simulink model "commhdlQPSKTxRxLoopback"  (R2025b)
settings: Solver=FixedStepDiscrete  StartTime=0.0  StopTime=0.03  RelTol=1e-3
PostLoadFcn:
  | hScopeConfig = get_param([gcs '/Receiver/QPSK Rx/Frequency and Time Synchronizer/Symbol Synchronizer/No HDL/QPSK Receiver Eye Diagram'],'ScopeConfiguration');
  | 
  | hScopeConfig.OpenAtSimulationStart = false;
  | hScopeConfig.Visible = false;
  | SamplesPerSymbol = 4;
  | %UpsamplesRx = 1;
  | clear hScopeConfig
InitFcn:
  | % RxAlign decoder latency (flat_simfix): 41 = netlist value used for HDL; set
  | % rxAlignLat = 25 in the base workspace before a model-level simulation.
  | if ~exist('rxAlignLat','var'), rxAlignLat = uint16(41); end
  | commhdlQPSKTxRxModelInit;
  | % Rate bridge: ADRV9002/Jupiter radio runs at 15.36 MHz = 2x the 7.68 MHz
  | % (4 samples/symbol @ Rsym=1.92 MHz) the QPSK Rx requires. The deployed
  | % Receiver must downsample the ADC stream by 2. UpsamplesRx=1 fed the QPSK
  | % Rx 8 sps (2x-upsampled) and broke symbol sync / the loopback bit check.
  | UpsamplesRx = 1;   %% T8 RATE FIX: rail 15.36e6 == ADC bus rate,
  | %% no ingress decimation (was 2 when the rail sat on the 7.68e6 rung)
  | UpsamplesTx = 1;
  | clear simTimingOffset;
StopFcn:
  | if exist('simTimingOffset','var')
  |   disp('Simulation completed');
  |   %QPSKTxRxVerification;
  | end
undefined symbols (not defined in the file or in its folder): Add, Config, fsym, randsrc, RandStream, Rsym, rxAlignLat, Shift
libraries: hdlsllib x141, simulink x45, dspsigops x30, dsphdlfiltering2 x6, dsphdlsigops2 x4, dsphdlmathfun2 x4, commdigbbndpm3 x4, dspmlti4 x2, commchan3 x1, commrflib2 x1, commcnvcod2 x1
(part 2 of 9)

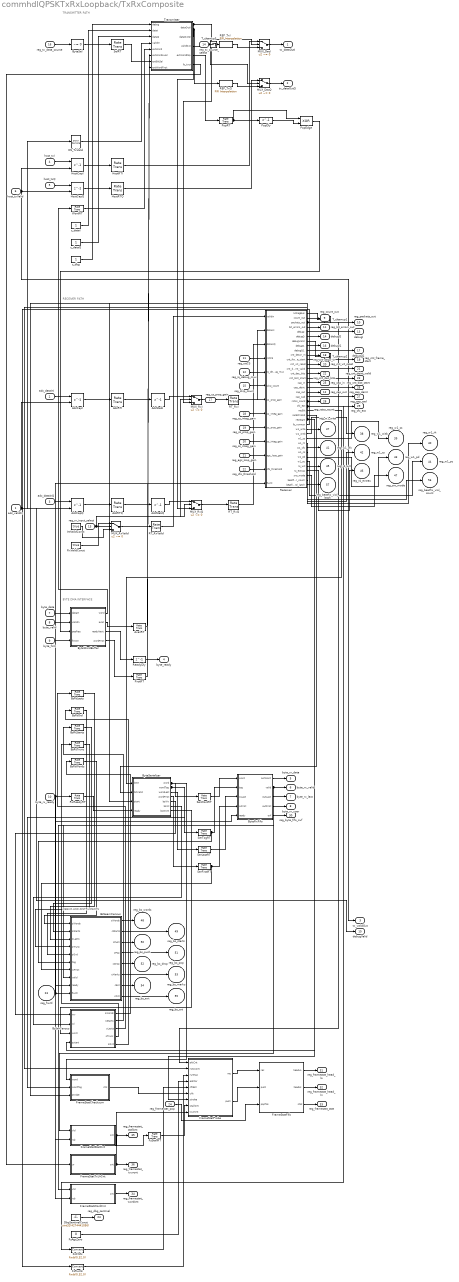
== system commhdlQPSKTxRxLoopback/TxRxComposite ==
  note: TRANSMITTER PATH
  note: RECEIVER PATH
  note: BYTE DMA INTERFACE
  note: DEBUG AND INSTRUMENTS
  adc_validIn : Inport  OutDataTypeStr=boolean  SampleTime=1/30.72e6
  adc_dataInI : Inport  Port=2  OutDataTypeStr=int16  SampleTime=1/30.72e6
  adc_dataInQ : Inport  Port=3  OutDataTypeStr=int16  SampleTime=1/30.72e6
  host_txI : Inport  Port=4  OutDataTypeStr=int16  SampleTime=1/30.72e6
  host_txQ : Inport  Port=5  OutDataTypeStr=int16  SampleTime=1/30.72e6
  host_txValid : Inport  Port=6  OutDataTypeStr=boolean  SampleTime=1/30.72e6
  byte_data : Inport  Port=7  OutDataTypeStr=uint64  SampleTime=1/30.72e6
  byte_valid : Inport  Port=8  OutDataTypeStr=boolean  SampleTime=1/30.72e6
  byte_first : Inport  Port=9  OutDataTypeStr=boolean  SampleTime=1/30.72e6
  byte_rx_ready : Inport  Port=10  OutDataTypeStr=boolean  SampleTime=1/30.72e6
  reg_rstCS : Inport  Port=11  OutDataTypeStr=boolean  SampleTime=1/15.36e6
  reg_iq_debug_mux : Inport  Port=12  OutDataTypeStr=uint32  SampleTime=1/15.36e6
  reg_rx_input_select : Inport  Port=13  OutDataTypeStr=boolean  SampleTime=1/15.36e6
  reg_tx_source_select : Inport  Port=14  OutDataTypeStr=uint32  SampleTime=1/15.36e6
  reg_skip_count : Inport  Port=15  OutDataTypeStr=uint32  SampleTime=1/15.36e6
  reg_tx_data_source : Inport  Port=16  OutDataTypeStr=uint32  SampleTime=1/15.36e6
  reg_cs_prop_gain : Inport  Port=17  OutDataTypeStr=uint32  SampleTime=1/15.36e6
  reg_cs_integ_gain : Inport  Port=18  OutDataTypeStr=uint32  SampleTime=1/15.36e6
  reg_ss_prop_gain : Inport  Port=19  OutDataTypeStr=uint32  SampleTime=1/15.36e6
  reg_ss_integ_gain : Inport  Port=20  OutDataTypeStr=uint32  SampleTime=1/15.36e6
  reg_agc_loop_gain : Inport  Port=21  OutDataTypeStr=uint32  SampleTime=1/15.36e6
  reg_cfo_threshold : Inport  Port=22  OutDataTypeStr=uint32  SampleTime=1/15.36e6
  reg_fixctl : Inport  Port=23  OutDataTypeStr=uint32
  reg_framestat_pop : Inport  Port=24  OutDataTypeStr=uint32  SampleTime=1/15.36e6
  AdcCapI : Delay  DelayLength=1  ShowEnablePort=on
      settings: InputPortMap=u0,e6
  AdcCapQ : Delay  DelayLength=1  ShowEnablePort=on
      settings: InputPortMap=u0,e6
  AdcRTI : RateTransition  OutPortSampleTime=1/15.36e6
  AdcRTQ : RateTransition  OutPortSampleTime=1/15.36e6
  AdcStabI : Delay  DelayLength=1
  AdcStabQ : Delay  DelayLength=1
  AvailRT : RateTransition  OutPortSampleTime=1/15.36e6
  BsRtLasts : RateTransition  OutPortSampleTime=1/30.72e6
  BsRtOrd : RateTransition  OutPortSampleTime=1/30.72e6
  BsRtStarts : RateTransition  OutPortSampleTime=1/30.72e6
  BsRtTrunc : RateTransition  OutPortSampleTime=1/30.72e6
  BsRtWords : RateTransition  OutPortSampleTime=1/30.72e6
  BsSeamCensus : MATLAB Function  TreatAsAtomicUnit=on
  BsSerCensus : MATLAB Function  TreatAsAtomicUnit=on
  ByteRxFifo : MATLAB Function  TreatAsAtomicUnit=on
  ByteSel : simulink/Logic and Bit Operations/Compare To Constant  relop=~=  const=0  OutDataTypeStr=boolean
  ByteSerializer : MATLAB Function  TreatAsAtomicUnit=on
  ByteWordBuffer : MATLAB Function  TreatAsAtomicUnit=on
  DS_TxValid : DownSample  N=1  RateOptions=Allow multirate processing  AllowArbitraryFixedInput=on
  DbgSentinelConst : Constant  Value=uint32(4274441056)  OutDataTypeStr=uint32  SampleTime=1/15.36e6
  FirstRT : RateTransition  OutPortSampleTime=1/15.36e6
  FrameStatChecksum : MATLAB Function  TreatAsAtomicUnit=on
  FrameStatFifo : MATLAB Function  TreatAsAtomicUnit=on
  FrameStatProbe : MATLAB Function  TreatAsAtomicUnit=on
  FrameStatStallCnt : MATLAB Function  TreatAsAtomicUnit=on
  FrameStatTxUrCnt : MATLAB Function  TreatAsAtomicUnit=on
  FrameStatWordCnt : MATLAB Function  TreatAsAtomicUnit=on
  FsAgcZero : Constant  Value=0  OutDataTypeStr=uint32
  FsCfcSi : DataTypeConversion  OutDataTypeStr=fixdt(0,32,0)  ConvertRealWorld=Stored Integer (SI)  SaturateOnIntegerOverflow=off  RndMeth=Floor
  FsRunSi : DataTypeConversion  OutDataTypeStr=fixdt(0,32,0)  ConvertRealWorld=Stored Integer (SI)  SaturateOnIntegerOverflow=off  RndMeth=Floor
  FsStallRT : RateTransition  OutPortSampleTime=1/15.36e6
  HostCapI : Delay  DelayLength=1  ShowEnablePort=on
      settings: InputPortMap=u0,e6
  HostCapQ : Delay  DelayLength=1  ShowEnablePort=on
      settings: InputPortMap=u0,e6
  HostRTI : RateTransition  OutPortSampleTime=1/30.72e6
  HostRTQ : RateTransition  OutPortSampleTime=1/30.72e6
  IntValidConst : Constant  Value=true  OutDataTypeStr=boolean  SampleTime=1/15.36e6
  MUX_DacI : Switch  Criteria=u2 ~= 0
  MUX_DacQ : Switch  Criteria=u2 ~= 0
  MUX_RxI : Switch  Criteria=u2 ~= 0
  MUX_RxQ : Switch  Criteria=u2 ~= 0
  MUX_RxValid : Switch  Criteria=u2 ~= 0
  PopDly : Delay  DelayLength=1
  PopEdge : Logic  Operator=XOR
  PopRT : RateTransition  OutPortSampleTime=1/30.72e6
  REP_TxI : dspmlti4/FIR Interpolation  FilterSource=Dialog parameters  PrivateCoeffs=0  h=2*fir1(24,0.45)  L=2  FilterObject=FINTERP  framing=Allow multirate processing  outputBufInitCond=0  roundingMode=Nearest  overflowMode=on  firstCoeffDataTypeStr=Inherit: Same word length as input  firstCoeffMin=[]  firstCoeffMax=[]  firstCoeffLastDataTypeStr=Inherit: Same word length as input  outputMin=[]  outputMax=[]
  REP_TxQ : dspmlti4/FIR Interpolation  FilterSource=Dialog parameters  PrivateCoeffs=0  h=2*fir1(24,0.45)  L=2  FilterObject=FINTERP  framing=Allow multirate processing  outputBufInitCond=0  roundingMode=Nearest  overflowMode=on  firstCoeffDataTypeStr=Inherit: Same word length as input  firstCoeffMin=[]  firstCoeffMax=[]  firstCoeffLastDataTypeStr=Inherit: Same word length as input  outputMin=[]  outputMax=[]
  RT_RxI : RateTransition  OutPortSampleTime=1/15.36e6
  RT_RxQ : RateTransition  OutPortSampleTime=1/15.36e6
  RT_RxValid : RateTransition  OutPortSampleTime=1/15.36e6
  ReadyDly : Delay  DelayLength=1  InitialCondition=1
  Receiver : Subsystem  TreatAsAtomicUnit=on
  RxReadyRT : RateTransition  OutPortSampleTime=1/15.36e6
  RxValidConst : Constant  Value=true  OutDataTypeStr=boolean  SampleTime=1/15.36e6
  SelRT : RateTransition  OutPortSampleTime=1/15.36e6
  SerFirstRT : RateTransition  OutPortSampleTime=1/30.72e6
  SerLastRT : RateTransition  OutPortSampleTime=1/30.72e6
  SerTogRT : RateTransition  OutPortSampleTime=1/30.72e6
  SerWordRT : RateTransition  OutPortSampleTime=1/30.72e6
  T_cleanup1 : Terminator
  T_cleanup2 : Terminator
  T_cleanup3 : Terminator
  Transmitter : Subsystem  TreatAsAtomicUnit=on
  WordRT : RateTransition  OutPortSampleTime=1/15.36e6
  c_dataI : Constant  OutDataTypeStr=int16  SampleTime=1/15.36e6
  c_dataQ : Constant  OutDataTypeStr=int16  SampleTime=1/15.36e6
  c_dbg : Constant  OutDataTypeStr=uint32  SampleTime=1/15.36e6
  tx_dataOutI : Outport
  tx_dataOutQ : Outport  Port=2
  tx_validOut : Outport  Port=3
  byte_ready : Outport  Port=4
  byte_rx_data : Outport  Port=5
  byte_rx_valid : Outport  Port=6
  byte_rx_last : Outport  Port=7
  byte_rx_user : Outport  Port=8
  reg_count_out : Outport  Port=9
  reg_packets_out : Outport  Port=10
  reg_bit_errors_out : Outport  Port=11
  reg_cap_out : Outport  Port=12
  debugI : Outport  Port=13
  debugQ : Outport  Port=14
  debugValid : Outport  Port=15
  debugI1 : Outport  Port=16
  debugQ1 : Outport  Port=17
  reg_cnt_descr_in : Outport  Port=18
  reg_cnt_frame_start : Outport  Port=19
  reg_cnt_vit_reset : Outport  Port=20
  reg_cnt_deint_valid : Outport  Port=21
  reg_cnt_dec_bits : Outport  Port=22
  reg_cnt_bist_start : Outport  Port=23
  reg_dbg_sentinel : Outport  Port=24
  reg_cap_in : Outport  Port=25
  reg_cap_deint : Outport  Port=26
  reg_cap_cad : Outport  Port=27
  reg_rstcs_count : Outport  Port=28
  reg_cfc_est : Outport  Port=29
  reg_byte_fifo_ovf : Outport  Port=30
  reg_framestat_head_lo : Outport  Port=31
  reg_framestat_head_hi : Outport  Port=32
  reg_framestat_stat : Outport  Port=33
  reg_framestat_wordcnt : Outport  Port=34
  reg_framestat_stallcnt : Outport  Port=35
  reg_framestat_txurcnt : Outport  Port=36
  reg_w1_wita : Outport  Port=37
  reg_w1_witb : Outport  Port=38
  reg_w1_ss : Outport  Port=39
  reg_w1_rh : Outport  Port=40
  reg_w1_cfc : Outport  Port=41
  reg_w1_cs : Outport  Port=42
  reg_w1_pd : Outport  Port=43
  reg_w1_pc : Outport  Port=44
  reg_r4_wit : Outport  Port=45
  reg_r4_extras : Outport  Port=46
  reg_sro_mode : Outport  Port=47
  reg_bs_words : Outport  Port=48
  reg_bs_starts : Outport  Port=49
  reg_bs_push : Outport  Port=50
  reg_bs_pop : Outport  Port=51
  reg_bs_drop : Outport  Port=52
  reg_bs_marks : Outport  Port=53
  reg_bs_evt : Outport  Port=54
  reg_bs_cnt : Outport  Port=55
  reg_beatfix_viol_count : Outport  Port=56
  reg_beatfix_viol_latch : Outport  Port=57
  wires:
  Receiver/30(w1_cfc) -> reg_w1_cfc/1
  BsSeamCensus/5(cDrop) -> reg_bs_drop/1
  FrameStatProbe/1(rec) -> FrameStatFifo/1(rec)
  host_txI/1 -> HostCapI/1
  MUX_RxValid/1 -> RT_RxValid/1
  Receiver/23(recBitValid) -> ByteSerializer/2(bitValid)
  byte_first/1 -> ByteWordBuffer/4(firstIn)
  AdcCapI/1 -> AdcRTI/1
  ByteSerializer/2(wordTog) -> FrameStatChecksum/2(wordTog), SerTogRT/1
  c_dataQ/1 -> Transmitter/3(dataQ)
  ByteRxFifo/3(outLast) -> byte_rx_last/1
  ReadyDly/1 -> byte_ready/1
  ByteRxFifo/5(ovf) -> reg_byte_fifo_ovf/1
  host_txValid/1 -> HostCapQ/2, HostCapI/2, tx_validOut/1
  BsRtTrunc/1 -> BsSeamCensus/4(sTrunc)
  DbgSentinelConst/1 -> reg_dbg_sentinel/1
  MUX_DacQ/1 -> tx_dataOutQ/1
  BsSeamCensus/4(cPop) -> reg_bs_pop/1
  AdcStabI/1 -> MUX_RxI/1
  BsSeamCensus/8(cCnt) -> reg_bs_cnt/1
  reg_tx_data_source/1 -> ByteSel/1
  AvailRT/1 -> Transmitter/6(extWordAvail)
  IntValidConst/1 -> MUX_RxValid/3
  Receiver/9(debugQ1) -> debugQ1/1
  adc_dataInI/1 -> AdcCapI/1
  ByteSerializer/3(wordLast) -> SerLastRT/1
  SerWordRT/1 -> ByteRxFifo/1(word)
  FrameStatWordCnt/1(cnt) -> reg_framestat_wordcnt/1
  Receiver/33(w1_pc) -> reg_w1_pc/1
  Receiver/29(w1_rh) -> reg_w1_rh/1
  reg_cs_integ_gain/1 -> Receiver/8(cs_integ_gain)
  Receiver/4(bit_errors_out) -> reg_bit_errors_out/1
  MUX_RxI/1 -> RT_RxI/1
  REP_TxI/1 -> MUX_DacI/3
  AdcRTQ/1 -> AdcStabQ/1
  Receiver/11(cnt_frame_start) -> reg_cnt_frame_start/1
  FrameStatTxUrCnt/1(cnt) -> reg_framestat_txurcnt/1, FrameStatProbe/9(txurCnt)
  Receiver/14(cnt_dec_bits) -> reg_cnt_dec_bits/1
  RT_RxI/1 -> Receiver/2(dataInI)
  Receiver/24(recStart) -> BsSerCensus/4(sstart), ByteSerializer/3(start), FrameStatProbe/7(strobe), FrameStatChecksum/3(strobe)
  Receiver/37(beatfix_viol_count) -> reg_beatfix_viol_count/1
  PopEdge/1 -> ByteWordBuffer/3(popReq)
  FrameStatFifo/1(headLo) -> reg_framestat_head_lo/1
  Receiver/38(beatfix_viol_latch) -> reg_beatfix_viol_latch/1
  Receiver/8(debugI1) -> debugI1/1
  Receiver/19(cap_cad) -> reg_cap_cad/1
  Receiver/15(cnt_bist_start) -> reg_cnt_bist_start/1
  BsSeamCensus/2(cStarts) -> reg_bs_starts/1
  byte_valid/1 -> ByteWordBuffer/2(validIn)
  reg_ss_prop_gain/1 -> Receiver/9(ss_prop_gain)
  HostRTQ/1 -> MUX_DacQ/1
  HostCapQ/1 -> HostRTQ/1
  Transmitter/4(extWordPop) -> PopRT/1
  BsSerCensus/3(sLasts) -> BsRtLasts/1
  Receiver/17(cap_deint) -> reg_cap_deint/1
  Receiver/21(cfc_est) -> FsCfcSi/1, reg_cfc_est/1
  BsSerCensus/1(sWords) -> BsRtWords/1
  MUX_RxQ/1 -> RT_RxQ/1
  Receiver/6(debugQ) -> debugQ/1
  Transmitter/1(dataOutI) -> REP_TxI/1, MUX_RxI/3
  RxValidConst/1 -> MUX_RxValid/1
  FrameStatChecksum/1(chk) -> FrameStatProbe/6(chk)
  SerTogRT/1 -> ByteRxFifo/2(tog), BsSeamCensus/6(tog)
  Receiver/34(r4_wit) -> reg_r4_wit/1
  Receiver/16(cap_in) -> reg_cap_in/1
  Receiver/31(w1_cs) -> reg_w1_cs/1
  ByteSel/1 -> SelRT/1
  Receiver/22(recBit) -> ByteSerializer/1(bitIn)
  Receiver/18(cap_out) -> reg_cap_out/1
  Receiver/26(w1_wita) -> reg_w1_wita/1
  DS_TxValid/1 -> Transmitter/4(validIn)
  ByteSerializer/6(bsWl) -> BsSerCensus/2(wl)
  FsCfcSi/1 -> FrameStatProbe/5(cfcEst)
  ByteSerializer/4(wordFirst) -> SerFirstRT/1
  FrameStatStallCnt/1(cnt) -> reg_framestat_stallcnt/1, FsStallRT/1
  FirstRT/1 -> Transmitter/8(extWordFirst)
  RT_RxQ/1 -> Receiver/3(dataInQ)
  Receiver/27(w1_witb) -> reg_w1_witb/1
  Receiver/3(packets_out) -> FrameStatProbe/1(pktCnt), reg_packets_out/1
  Receiver/10(cnt_descr_in) -> reg_cnt_descr_in/1
  reg_ss_integ_gain/1 -> Receiver/10(ss_integ_gain)
  Receiver/2(count_out) -> reg_count_out/1
  reg_skip_count/1 -> Receiver/6(skip_count)
  byte_rx_ready/1 -> RxReadyRT/1, FrameStatWordCnt/2(rdy), ByteRxFifo/5(ready), FrameStatStallCnt/2(rdy), BsSeamCensus/9(ready)
  SerFirstRT/1 -> ByteRxFifo/4(wFirst), BsSeamCensus/7(wFirst)
  HostCapI/1 -> HostRTI/1
  BsRtOrd/1 -> BsSeamCensus/5(sOrd)
  adc_dataInQ/1 -> AdcCapQ/1
  Receiver/32(w1_pd) -> reg_w1_pd/1
  reg_cs_prop_gain/1 -> Receiver/7(cs_prop_gain)
  PopRT/1 -> PopDly/1, PopEdge/1
  BsSerCensus/2(sStarts) -> BsRtStarts/1
  Receiver/20(rstcs_count) -> reg_rstcs_count/1, FrameStatProbe/2(rstcsCnt)
  FsRunSi/1 -> FrameStatProbe/3(runMax)
  reg_fixctl/1 -> BsSeamCensus/10(fixctl), Receiver/13(fixctl)
  BsRtWords/1 -> BsSeamCensus/1(sWords)
  FrameStatProbe/2(push) -> FrameStatFifo/2(push)
  BsSeamCensus/3(cPush) -> reg_bs_push/1
  MUX_DacI/1 -> tx_dataOutI/1
  SelRT/1 -> Transmitter/7(extBitSel)
  reg_framestat_pop/1 -> FrameStatFifo/3(popTok)
  FrameStatFifo/2(headHi) -> reg_framestat_head_hi/1
  Receiver/35(r4_extras) -> reg_r4_extras/1
  ByteRxFifo/4(outFirst) -> byte_rx_user/1
  REP_TxQ/1 -> MUX_DacQ/3
  reg_cfo_threshold/1 -> Receiver/12(cfo_threshold)
  Receiver/25(fs_runmax) -> FsRunSi/1
  Receiver/12(cnt_vit_reset) -> reg_cnt_vit_reset/1
  reg_agc_loop_gain/1 -> Receiver/11(agc_loop_gain)
  Transmitter/2(dataOutQ) -> REP_TxQ/1, MUX_RxQ/3
  reg_tx_source_select/1 -> MUX_DacI/2, MUX_DacQ/2
  RxReadyRT/1 -> ByteSerializer/4(ready)
  Transmitter/5(fs_txur) -> FrameStatTxUrCnt/1(ur)
  reg_rstCS/1 -> Receiver/4(rstCS)
  SerLastRT/1 -> ByteRxFifo/3(wLast)
  BsRtStarts/1 -> BsSeamCensus/2(sStarts)
  BsSeamCensus/7(cEvt) -> reg_bs_evt/1
  PopDly/1 -> PopEdge/2
  BsRtLasts/1 -> BsSeamCensus/3(sLasts)
  host_txQ/1 -> HostCapQ/1
  ByteSerializer/7(bsWcnt) -> BsSerCensus/3(wcnt)
  c_dbg/1 -> Transmitter/1(debug)
  Receiver/5(debugI) -> debugI/1
  BsSeamCensus/1(cWords) -> reg_bs_words/1
  ByteRxFifo/2(valid) -> byte_rx_valid/1, BsSeamCensus/8(valid), FrameStatWordCnt/1(vld), FrameStatStallCnt/1(vld)
  byte_data/1 -> ByteWordBuffer/1(dataIn)
  FrameStatFifo/3(stat) -> reg_framestat_stat/1
  reg_iq_debug_mux/1 -> Receiver/5(iq_debug_mux)
  WordRT/1 -> Transmitter/5(extWord)
  ByteWordBuffer/4(wordFirst) -> FirstRT/1
  ByteSerializer/1(word) -> FrameStatChecksum/1(word), SerWordRT/1
  ByteRxFifo/1(outWord) -> byte_rx_data/1
  ByteSerializer/5(bsWv) -> BsSerCensus/1(wv)
  BsSerCensus/5(sOrd) -> BsRtOrd/1
  ByteWordBuffer/2(avail) -> AvailRT/1
  RT_RxValid/1 -> Receiver/1(validIn)
  BsSeamCensus/6(cMarks) -> reg_bs_marks/1
  adc_validIn/1 -> debugValid/1, AdcCapQ/2, DS_TxValid/1, AdcCapI/2
  HostRTI/1 -> MUX_DacI/1
  BsSerCensus/4(sTrunc) -> BsRtTrunc/1
  Receiver/36(sro_mode) -> reg_sro_mode/1
  ByteWordBuffer/1(word) -> WordRT/1
  reg_rx_input_select/1 -> MUX_RxValid/2, MUX_RxQ/2, MUX_RxI/2
  FsAgcZero/1 -> FrameStatProbe/4(adcFor)
  AdcRTI/1 -> AdcStabI/1
  AdcStabQ/1 -> MUX_RxQ/1
  ByteWordBuffer/3(readyNext) -> ReadyDly/1
  Receiver/28(w1_ss) -> reg_w1_ss/1
  AdcCapQ/1 -> AdcRTQ/1
  FsStallRT/1 -> FrameStatProbe/8(stallCnt)
  Receiver/13(cnt_deint_valid) -> reg_cnt_deint_valid/1
  c_dataI/1 -> Transmitter/2(dataI)
  Receiver/1(rxDiagBus) -> T_cleanup1/1
  Receiver/7(debugValid) -> T_cleanup2/1
  Transmitter/3(validOut) -> T_cleanup3/1

== system commhdlQPSKTxRxLoopback/Capture Tx Diagnostics/Subsystem ==
  In1 : Inport
  Enable : EnablePort
  To Workspace : ToWorkspace  VariableName=simQPSKSym  SampleTime=-1
      settings: Save2DSignal=2-D array (concatenate along first dimension)
  wires:
  In1/1 -> To Workspace/1

== system commhdlQPSKTxRxLoopback/Capture Tx Diagnostics/Subsystem1 ==
  In1 : Inport
  Enable : EnablePort
  To Workspace1 : ToWorkspace  VariableName=simTxWaveform  SampleTime=-1
      settings: Save2DSignal=2-D array (concatenate along first dimension)
  wires:
  In1/1 -> To Workspace1/1

== system commhdlQPSKTxRxLoopback/Channel/Mod 1 ==
  In1 : Inport
  Constant : Constant  SampleTime=-1
  Mod : Math  Operator=mod
  Out1 : Outport
  wires:
  Mod/1 -> Out1/1
  In1/1 -> Mod/1
  Constant/1 -> Mod/2

== system commhdlQPSKTxRxLoopback/Receiver/Capture Data Bits ==
  dataOut : Inport
  dataSrt : Inport  Port=2
  dataEnd : Inport  Port=3
  valid : Inport  Port=4
  Display : Display
  Display1 : Display
  Display2 : Display
  MATLAB Function : MATLAB Function  TreatAsAtomicUnit=on
  To Workspace : ToWorkspace  VariableName=RxOut  SampleTime=-1
      settings: Save2DSignal=2-D array (concatenate along first dimension)
  To Workspace1 : ToWorkspace  VariableName=RxOutSrt  SampleTime=-1
      settings: Save2DSignal=2-D array (concatenate along first dimension)
  To Workspace2 : ToWorkspace  VariableName=RxOutEnd  SampleTime=-1
      settings: Save2DSignal=2-D array (concatenate along first dimension)
  count_out : Outport
  packets_out : Outport  Port=2
  bit_errors_out : Outport  Port=3
  wires:
  dataOut/1 -> MATLAB Function/2(datain), To Workspace/1
  dataSrt/1 -> MATLAB Function/3(start), To Workspace1/1
  dataEnd/1 -> MATLAB Function/4(stop), To Workspace2/1
  valid/1 -> MATLAB Function/1(valid)
  MATLAB Function/1(count_out) -> count_out/1, Display/1
  MATLAB Function/2(packets_out) -> packets_out/1, Display1/1
  MATLAB Function/3(bit_errors_out) -> bit_errors_out/1, Display2/1

== system commhdlQPSKTxRxLoopback/Receiver/QPSK Rx ==
  dataIn : Inport  OutDataTypeStr=fixdt(1,16,14)  PortDimensions=1  SampleTime=1/(Rsym*SamplesPerSymbol)
      settings: SignalType=complex
  validIn : Inport  Port=2  OutDataTypeStr=boolean  PortDimensions=1  SampleTime=1/(Rsym*SamplesPerSymbol)
  rstCS : Inport  Port=3  OutDataTypeStr=boolean  PortDimensions=1
      settings: SignalType=complex
  debugMuxCtrl : Inport  Port=4  OutDataTypeStr=uint32  PortDimensions=1  SampleTime=1/(Rsym*SamplesPerSymbol)
  Automatic Gain Control : Subsystem  mask{Ref=AGCReference, LFG=AGCLoopGain}
      mask prompts: Ref "Error Detector Reference:"; LFG "Loop Filter Gain"
  Bus Creator : BusCreator  Inputs=4
  Bus Creator1 : BusCreator  Inputs=3
  Complex to Real-Imag : ComplexToRealImag
  Constant : Constant  Value=true  SampleTime=1/(Rsym*SamplesPerSymbol)
  Data Type Conversion : DataTypeConversion  OutDataTypeStr=int16  ConvertRealWorld=Stored Integer (SI)  SaturateOnIntegerOverflow=off  RndMeth=Floor
  Delay{,1..8} (9 alike) : Delay  DelayLength=1
  Frequency and Time Synchronizer : Subsystem
      settings: PortSchema="{\"entries\":[{\"content\":{\"sides\":[{\"content\":{\"connectorIds\":[\"In1\",\"In2\"]},\"type\":\"ConnectorPlacement.EquallySpacedRectSide\",\"uuid\":\"8bc6a452-5111-4806-8ca9-335cb622aea6\"},{\"content\":{\"connectorIds\":[\"Out1\",\"Out2\",\"Out3\",\"Out4\"],\"side\":\"RIGHT\"},\"type\":\"ConnectorPlacement.EquallySpacedRectSide\",\"uuid\":\"b0f43c98-f5c0-4f62-94ae-d69789942eef\"},{\"content\":{\"connectorIds\":[\"In3\",\"Out7\",\"Out8\"],\"side\":\"TOP\"},\"type\":\"ConnectorPlacement.EquallySpacedRectSide\",\"uuid\":\"427ff3b3-b896-4008-9584-d311480df763\"},{\"content\":{\"connectorIds\":[\"Out5\",\"Out6\"],\"side\":\"BOTTOM\"},\"type\":\"ConnectorPlacement.EquallySpacedRectSide\",\"uuid\":\"f704cb90-80a1-4198-8b72-e70182b45e73\"},{\"content\":{\"side\":\"HIDDEN\"},\"type\":\"ConnectorPlacement.EquallySpacedRectSide\",\"uuid\":\"f6309498-1e43-486f-b6b5-2c6570711f8e\"}]},\"type\":\"ConnectorPlacement.EquallySpacedConnector\",\"uuid\":\"f0ce492e-c9e1-4b35-98ef-84d77b696cfe\"}],\"packageUris\":[\"http://schema.mathworks.com/mf0/Connector/R2020b\"],\"version\":\"1.0\"}"
  HDL Data Descrambler : Subsystem
  Index Vector : MultiPortSwitch  DataPortOrder=Zero-based contiguous  Inputs=4  DiagnosticForDefault=None  zeroidx=on  SaturateOnIntegerOverflow=off  InputSameDT=off
  QPSK Demodulator : Subsystem
  RRC Receive Filter : dsphdlfiltering2/Discrete FIR Filter  NumeratorSource=Property  Numerator=RRCCoef  NumeratorPrototype=[]  FilterStructure=Direct form systolic  SerializationOption=Minimum number of cycles between valid input samples  NumCycles=2  NumberOfMultipliers=2  SimulateUsing=Code generation  roundingMode=Floor  overflowMode=off  CoefficientsDataTypeStr=Inherit: Same word length as input  OutputDataTypeStr=Inherit: Same word length as input  ResetInputPort=off  HDLGlobalReset=off  CoeffMultiplier=Multiplier  UseMultForPow2Coeff=on  FrameInputSymmOptim=off
  dataOut : Outport
  ctrlOut : Outport  Port=2
  rxDiagBus : Outport  Port=3
  debugIOut : Outport  Port=4
  debugQOut : Outport  Port=5
  debugValid : Outport  Port=6
  wires:
  rstCS/1 -> Frequency and Time Synchronizer/3(rstCS)
  QPSK Demodulator/1(dataOut) -> HDL Data Descrambler/1(dataIn)
  validIn/1 -> Automatic Gain Control/2(validIn)
  Automatic Gain Control/2(validOut) -> RRC Receive Filter/2
  RRC Receive Filter/1 -> Frequency and Time Synchronizer/1(dataIn)
  HDL Data Descrambler/3(endOut) -> Bus Creator1/2  "endOut"
  QPSK Demodulator/3(endOut) -> HDL Data Descrambler/3(endIn)
  Frequency and Time Synchronizer/8(normCoarseFreqEst) -> Bus Creator/2  "normCoarseFreqEst"
  Bus Creator1/1 -> ctrlOut/1
  HDL Data Descrambler/2(startOut) -> Bus Creator1/1  "startOut"
  Frequency and Time Synchronizer/3(endOut) -> QPSK Demodulator/3(endIn)
  RRC Receive Filter/2 -> Frequency and Time Synchronizer/2(validIn)
  Frequency and Time Synchronizer/7(nSynced) -> Bus Creator/1  "nSynced"
  Bus Creator/1 -> Delay/1
  Automatic Gain Control/1(dataOut) -> Delay1/1, RRC Receive Filter/1
  Frequency and Time Synchronizer/1(dataOut) -> Delay4/1, QPSK Demodulator/1(dataIn), Bus Creator/3  "QPSKConstellationPoints"
  dataIn/1 -> Automatic Gain Control/1(dataIn)
  HDL Data Descrambler/1(dataOut) -> dataOut/1
  HDL Data Descrambler/4(validOut) -> Bus Creator1/3  "validOut"
  QPSK Demodulator/2(startOut) -> HDL Data Descrambler/2(startIn)
  Frequency and Time Synchronizer/2(startOut) -> QPSK Demodulator/2(startIn)
  Frequency and Time Synchronizer/4(validOut) -> QPSK Demodulator/4(validIn), Bus Creator/4  "QPSKConstellationValid"
  QPSK Demodulator/4(validOut) -> HDL Data Descrambler/4(validIn)
  Delay/1 -> rxDiagBus/1
  Frequency and Time Synchronizer/5(postSymbolSync) -> Delay2/1
  Frequency and Time Synchronizer/6(postCarrierSync) -> Delay3/1
  debugMuxCtrl/1 -> Index Vector/1
  Complex to Real-Imag/2 -> debugQOut/1
  Complex to Real-Imag/1 -> debugIOut/1
  Data Type Conversion/1 -> Delay6/1
  Delay1/1 -> Index Vector/2
  Delay2/1 -> Index Vector/3
  Delay3/1 -> Index Vector/4
  Delay4/1 -> Index Vector/5
  Delay5/1 -> Data Type Conversion/1
  Index Vector/1 -> Delay5/1
  Delay6/1 -> Complex to Real-Imag/1
  Delay7/1 -> debugValid/1
  Delay8/1 -> Delay7/1
  Constant/1 -> Delay8/1

== system commhdlQPSKTxRxLoopback/Transmitter/Input Data ==
  enb : Inport
  reset : Inport  Port=2
  Cast To Boolean : DataTypeConversion  OutDataTypeStr=boolean  SaturateOnIntegerOverflow=off  RndMeth=Floor
  Delay : Delay  DelayLength=1
  Display : Display
  Message Generator : Subsystem
  Terminator : Terminator
  Terminator1 : Terminator
  txData : Outport
  txValid : Outport  Port=2
  msg_count_out : Outport  Port=3
  wires:
  Message Generator/4(valid) -> txValid/1
  Message Generator/1(out) -> txData/1
  enb/1 -> Message Generator/2(enable)
  Message Generator/5(count) -> Display/1
  Message Generator/2(stop) -> Delay/1
  Delay/1 -> Cast To Boolean/1
  Cast To Boolean/1 -> Message Generator/1(reset)
  reset/1 -> Terminator/1
  Message Generator/3(start) -> Terminator1/1
  Message Generator/6(msg_count_out) -> msg_count_out/1

== system commhdlQPSKTxRxLoopback/Transmitter/QPSK Tx ==
  dataIn : Inport  OutDataTypeStr=boolean  PortDimensions=1
  validIn : Inport  Port=2  OutDataTypeStr=boolean  PortDimensions=1
  Bit Packetizer : Subsystem
  Bus Creator : BusCreator  Inputs=2
  HDL Data Scrambler : Subsystem
  QPSK Modulator : Subsystem
  RRC Transmit Filter : Subsystem
  dataReady : Outport
  dataOut : Outport  Port=2
  txDiagBus : Outport  Port=3
  validOut : Outport  Port=4
  wires:
  validIn/1 -> Bit Packetizer/2(validIn)
  RRC Transmit Filter/2(validOut) -> validOut/1
  HDL Data Scrambler/1(dataOut) -> QPSK Modulator/1(dataIn)
  Bit Packetizer/1(bitsOut) -> HDL Data Scrambler/1(dataIn)
  QPSK Modulator/2(validOut) -> Bus Creator/2, RRC Transmit Filter/2(validIn)  "QPSKConstellationValid"
  dataIn/1 -> Bit Packetizer/1(dataIn)
  Bit Packetizer/3(dataEnd) -> HDL Data Scrambler/3(endIn)
  HDL Data Scrambler/2(validOut) -> QPSK Modulator/2(validIn)
  RRC Transmit Filter/1(dataOut) -> dataOut/1
  QPSK Modulator/1(dataOut) -> Bus Creator/1, RRC Transmit Filter/1(dataIn)  "QPSKConstellationPoints"
  Bit Packetizer/2(dataStart) -> HDL Data Scrambler/2(startIn)
  Bit Packetizer/5(dataReady) -> dataReady/1
  Bus Creator/1 -> txDiagBus/1
  Bit Packetizer/4(bitsValid) -> HDL Data Scrambler/4(validIn)

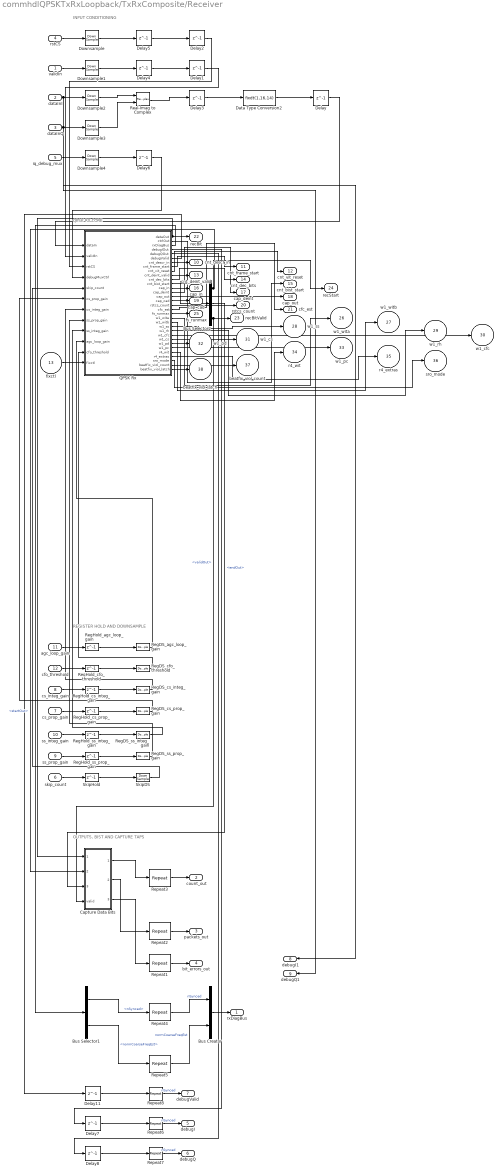
== system commhdlQPSKTxRxLoopback/TxRxComposite/Receiver ==
  note: INPUT CONDITIONING
  note: QPSK RX CORE
  note: REGISTER HOLD AND DOWNSAMPLE
  note: OUTPUTS, BIST AND CAPTURE TAPS
  validIn : Inport
  dataInI : Inport  Port=2
  dataInQ : Inport  Port=3
  rstCS : Inport  Port=4
  iq_debug_mux : Inport  Port=5  OutDataTypeStr=uint32
  skip_count : Inport  Port=6  OutDataTypeStr=uint32  SampleTime=1/15.36e6
  cs_prop_gain : Inport  Port=7  OutDataTypeStr=uint32  SampleTime=1/15.36e6
  cs_integ_gain : Inport  Port=8  OutDataTypeStr=uint32  SampleTime=1/15.36e6
  ss_prop_gain : Inport  Port=9  OutDataTypeStr=uint32  SampleTime=1/15.36e6
  ss_integ_gain : Inport  Port=10  OutDataTypeStr=uint32  SampleTime=1/15.36e6
  agc_loop_gain : Inport  Port=11  OutDataTypeStr=uint32  SampleTime=1/15.36e6
  cfo_threshold : Inport  Port=12  OutDataTypeStr=uint32  SampleTime=1/15.36e6
  fixctl : Inport  Port=13  OutDataTypeStr=uint32
  Bus Creator : BusCreator  Inputs=2
  Bus Selector1 : BusSelector  OutputSignals=nSynced,normCoarseFreqEst
  Bus Selector2 : BusSelector  OutputSignals=startOut,endOut,validOut
  Capture Data Bits : Subsystem
  Data Type Conversion2 : DataTypeConversion  OutDataTypeStr=fixdt(1,16,14)  ConvertRealWorld=Stored Integer (SI)  SaturateOnIntegerOverflow=off  RndMeth=Floor
  Delay{,1..8,11} (10 alike) : Delay  DelayLength=1
  Downsample{,1..4} (5 alike) : DownSample  N=UpsamplesRx  RateOptions=Allow multirate processing
  QPSK Rx : Subsystem
      mask init: same as commhdlQPSKTxRxLoopback/Receiver/QPSK Rx
  Real-Imag to Complex : RealImagToComplex
  RegDS_agc_loop_gain : DownSample  N=1  RateOptions=Allow multirate processing  AllowArbitraryFixedInput=on
  RegDS_cfo_threshold : DownSample  N=1  RateOptions=Allow multirate processing  AllowArbitraryFixedInput=on
  RegDS_cs_integ_gain : DownSample  N=1  RateOptions=Allow multirate processing  AllowArbitraryFixedInput=on
  RegDS_cs_prop_gain : DownSample  N=1  RateOptions=Allow multirate processing  AllowArbitraryFixedInput=on
  RegDS_ss_integ_gain : DownSample  N=1  RateOptions=Allow multirate processing  AllowArbitraryFixedInput=on
  RegDS_ss_prop_gain : DownSample  N=1  RateOptions=Allow multirate processing  AllowArbitraryFixedInput=on
  RegHold_agc_loop_gain : Delay  DelayLength=1
  RegHold_cfo_threshold : Delay  DelayLength=1
  RegHold_cs_integ_gain : Delay  DelayLength=1
  RegHold_cs_prop_gain : Delay  DelayLength=1
  RegHold_ss_integ_gain : Delay  DelayLength=1
  RegHold_ss_prop_gain : Delay  DelayLength=1
  Repeat{1..8} (8 alike) : dspsigops/Repeat  FactorSource=Dialog parameter  N=UpsamplesRx  Nmax=16  InputProcessing=Columns as channels (frame based)  RateOptions=Allow multirate processing  ic=0  mode=Unused parameter value
      settings: LibrarySourceBlock=commsequence2/Repeat
  SkipDS : DownSample  N=1  RateOptions=Allow multirate processing  AllowArbitraryFixedInput=on
  SkipHold : Delay  DelayLength=1
  rxDiagBus : Outport
  count_out : Outport  Port=2
  packets_out : Outport  Port=3
  bit_errors_out : Outport  Port=4
  debugI : Outport  Port=5
  debugQ : Outport  Port=6
  debugValid : Outport  Port=7
  debugI1 : Outport  Port=8
  debugQ1 : Outport  Port=9
  cnt_descr_in : Outport  Port=10
  cnt_frame_start : Outport  Port=11
  cnt_vit_reset : Outport  Port=12
  cnt_deint_valid : Outport  Port=13
  cnt_dec_bits : Outport  Port=14
  cnt_bist_start : Outport  Port=15
  cap_in : Outport  Port=16
  cap_deint : Outport  Port=17
  cap_out : Outport  Port=18
  cap_cad : Outport  Port=19
  rstcs_count : Outport  Port=20
  cfc_est : Outport  Port=21
  recBit : Outport  Port=22
  recBitValid : Outport  Port=23
  recStart : Outport  Port=24
  fs_runmax : Outport  Port=25
  w1_wita : Outport  Port=26
  w1_witb : Outport  Port=27
  w1_ss : Outport  Port=28
  w1_rh : Outport  Port=29
  w1_cfc : Outport  Port=30
  w1_cs : Outport  Port=31
  w1_pd : Outport  Port=32
  w1_pc : Outport  Port=33
  r4_wit : Outport  Port=34
  r4_extras : Outport  Port=35
  sro_mode : Outport  Port=36
  beatfix_viol_count : Outport  Port=37
  beatfix_viol_latch : Outport  Port=38
  wires:
  Downsample3/1 -> Real-Imag to Complex/2
  validIn/1 -> Downsample1/1
  Bus Selector2/1 -> Capture Data Bits/2(dataSrt), recStart/1  "<startOut>"
  Bus Selector2/2 -> Capture Data Bits/3(dataEnd)  "<endOut>"
  Bus Selector2/3 -> recBitValid/1, Capture Data Bits/4(valid)  "<validOut>"
  Delay3/1 -> Data Type Conversion2/1
  Delay1/1 -> QPSK Rx/2(validIn)
  Delay6/1 -> QPSK Rx/4(debugMuxCtrl)
  Downsample4/1 -> Delay6/1
  Capture Data Bits/1(count_out) -> Repeat3/1
  Capture Data Bits/2(packets_out) -> Repeat2/1
  Capture Data Bits/3(bit_errors_out) -> Repeat1/1
  Data Type Conversion2/1 -> Delay/1
  QPSK Rx/3(rxDiagBus) -> Bus Selector1/1
  QPSK Rx/1(dataOut) -> recBit/1, Capture Data Bits/1(dataOut)
  QPSK Rx/5(debugQOut) -> Delay8/1
  QPSK Rx/8(cnt_frame_start) -> cnt_frame_start/1
  QPSK Rx/9(cnt_vit_reset) -> cnt_vit_reset/1
  QPSK Rx/4(debugIOut) -> Delay7/1
  SkipDS/1 -> QPSK Rx/5(skip_count)
  RegHold_cfo_threshold/1 -> RegDS_cfo_threshold/1
  RegDS_cfo_threshold/1 -> QPSK Rx/11(cfo_threshold)
  QPSK Rx/21(w1_witb) -> w1_witb/1
  dataInQ/1 -> Downsample3/1, debugQ1/1
  QPSK Rx/14(cap_deint) -> cap_deint/1
  Bus Selector1/1 -> Repeat4/1  "<nSynced>"
  Repeat4/1 -> Bus Creator/1  "nSynced"
  iq_debug_mux/1 -> Downsample4/1
  RegHold_agc_loop_gain/1 -> RegDS_agc_loop_gain/1
  SkipHold/1 -> SkipDS/1
  RegHold_ss_prop_gain/1 -> RegDS_ss_prop_gain/1
  Bus Creator/1 -> rxDiagBus/1
  rstCS/1 -> Downsample/1
  cs_prop_gain/1 -> RegHold_cs_prop_gain/1
  Delay4/1 -> Delay1/1
  QPSK Rx/13(cap_in) -> cap_in/1
  Downsample/1 -> Delay5/1
  Delay/1 -> QPSK Rx/1(dataIn)
  ss_prop_gain/1 -> RegHold_ss_prop_gain/1
  cfo_threshold/1 -> RegHold_cfo_threshold/1
  QPSK Rx/20(w1_wita) -> w1_wita/1
  Delay7/1 -> Repeat6/1
  skip_count/1 -> SkipHold/1
  RegHold_ss_integ_gain/1 -> RegDS_ss_integ_gain/1
  QPSK Rx/22(w1_ss) -> w1_ss/1
  QPSK Rx/2(ctrlOut) -> Bus Selector2/1
  Delay8/1 -> Repeat7/1
  Delay5/1 -> Delay2/1
  Bus Selector1/2 -> Repeat5/1  "<normCoarseFreqEst>"
  QPSK Rx/12(cnt_bist_start) -> cnt_bist_start/1
  cs_integ_gain/1 -> RegHold_cs_integ_gain/1
  ss_integ_gain/1 -> RegHold_ss_integ_gain/1
  Repeat5/1 -> Bus Creator/2  "normCoarseFreqEst"
  Repeat8/1 -> debugValid/1  "nSynced"
  QPSK Rx/10(cnt_deint_valid) -> cnt_deint_valid/1
  RegHold_cs_integ_gain/1 -> RegDS_cs_integ_gain/1
  RegDS_cs_integ_gain/1 -> QPSK Rx/7(cs_integ_gain)
  RegDS_ss_prop_gain/1 -> QPSK Rx/8(ss_prop_gain)
  agc_loop_gain/1 -> RegHold_agc_loop_gain/1
  Repeat6/1 -> debugI/1  "nSynced"
  RegDS_cs_prop_gain/1 -> QPSK Rx/6(cs_prop_gain)
  QPSK Rx/29(r4_extras) -> r4_extras/1
  QPSK Rx/7(cnt_descr_in) -> cnt_descr_in/1
  fixctl/1 -> QPSK Rx/12(fixctl)
  RegDS_agc_loop_gain/1 -> QPSK Rx/10(agc_loop_gain)
  dataInI/1 -> debugI1/1, Downsample2/1
  Real-Imag to Complex/1 -> Delay3/1
  RegDS_ss_integ_gain/1 -> QPSK Rx/9(ss_integ_gain)
  QPSK Rx/31(beatfix_viol_count) -> beatfix_viol_count/1
  RegHold_cs_prop_gain/1 -> RegDS_cs_prop_gain/1
  QPSK Rx/11(cnt_dec_bits) -> cnt_dec_bits/1
  QPSK Rx/6(debugValid) -> Delay11/1
  Repeat3/1 -> count_out/1
  Downsample2/1 -> Real-Imag to Complex/1
  QPSK Rx/32(beatfix_viol_latch) -> beatfix_viol_latch/1
  Repeat2/1 -> packets_out/1
  Repeat7/1 -> debugQ/1  "nSynced"
  QPSK Rx/30(sro_mode) -> sro_mode/1
  Delay2/1 -> QPSK Rx/3(rstCS)
  QPSK Rx/28(r4_wit) -> r4_wit/1
  QPSK Rx/18(cfc_est) -> cfc_est/1
  QPSK Rx/27(w1_pc) -> w1_pc/1
  QPSK Rx/26(w1_pd) -> w1_pd/1
  Repeat1/1 -> bit_errors_out/1
  QPSK Rx/19(fs_runmax) -> fs_runmax/1
  QPSK Rx/17(rstcs_count) -> rstcs_count/1
  Delay11/1 -> Repeat8/1
  QPSK Rx/25(w1_cs) -> w1_cs/1
  QPSK Rx/16(cap_cad) -> cap_cad/1
  QPSK Rx/24(w1_cfc) -> w1_cfc/1
  QPSK Rx/23(w1_rh) -> w1_rh/1
  Downsample1/1 -> Delay4/1
  QPSK Rx/15(cap_out) -> cap_out/1

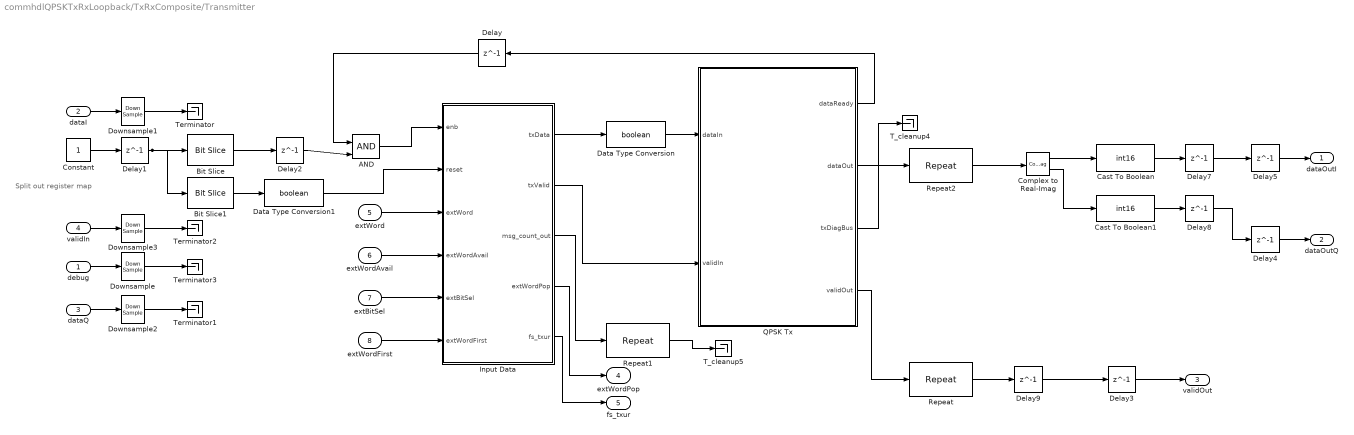
== system commhdlQPSKTxRxLoopback/TxRxComposite/Transmitter ==
  note: Split out register map
  debug : Inport  PortDimensions=1
  dataI : Inport  Port=2
  dataQ : Inport  Port=3
  validIn : Inport  Port=4
  extWord : Inport  Port=5  OutDataTypeStr=uint64
  extWordAvail : Inport  Port=6  OutDataTypeStr=boolean
  extBitSel : Inport  Port=7  OutDataTypeStr=boolean
  extWordFirst : Inport  Port=8  OutDataTypeStr=boolean
  AND : Logic  IconShape=distinctive  AllPortsSameDT=off  OutDataTypeStr=boolean
  Bit Slice : hdlsllib/Logic and Bit Operations/Bit Slice  lidx=0  ridx=0
  Bit Slice1 : hdlsllib/Logic and Bit Operations/Bit Slice  lidx=1  ridx=1
  Cast To Boolean : DataTypeConversion  OutDataTypeStr=int16  ConvertRealWorld=Stored Integer (SI)  SaturateOnIntegerOverflow=off  RndMeth=Floor
  Cast To Boolean1 : DataTypeConversion  OutDataTypeStr=int16  ConvertRealWorld=Stored Integer (SI)  SaturateOnIntegerOverflow=off  RndMeth=Floor
  Complex to Real-Imag : ComplexToRealImag
  Constant : Constant  OutDataTypeStr=uint32  SampleTime=-1
  Data Type Conversion : DataTypeConversion  OutDataTypeStr=boolean  SaturateOnIntegerOverflow=off  RndMeth=Floor
  Data Type Conversion1 : DataTypeConversion  OutDataTypeStr=boolean  SaturateOnIntegerOverflow=off  RndMeth=Floor
  Delay{,1..5,7..9} (9 alike) : Delay  DelayLength=1
  Downsample{,1..3} (4 alike) : DownSample  N=UpsamplesTx  RateOptions=Allow multirate processing
  Input Data : Subsystem  mask{dataBits=reshape(repmat(randsrc(2240*1,1,[0,1],RandStream('mcg16807','Seed',0)), 59,1), [2240*59,1]), Rsym=7.68e6}
      mask prompts: dataBits "Data Bits :"; Rsym "Symbol Rate (in baud rate)  :"
      mask Display: disp(['Double-Click' newline 'to set data bits']);
  QPSK Tx : Subsystem
      mask init: same as commhdlQPSKTxRxLoopback/Transmitter/QPSK Tx
  Repeat : dspsigops/Repeat  FactorSource=Dialog parameter  N=UpsamplesTx  Nmax=16  InputProcessing=Columns as channels (frame based)  RateOptions=Allow multirate processing  ic=0  mode=Unused parameter value
      settings: LibrarySourceBlock=commsequence2/Repeat
  Repeat1 : dspsigops/Repeat  FactorSource=Dialog parameter  N=UpsamplesTx  Nmax=16  InputProcessing=Columns as channels (frame based)  RateOptions=Allow multirate processing  ic=0  mode=Unused parameter value
      settings: LibrarySourceBlock=commsequence2/Repeat
  Repeat2 : dspsigops/Repeat  FactorSource=Dialog parameter  N=UpsamplesTx  Nmax=16  InputProcessing=Columns as channels (frame based)  RateOptions=Allow multirate processing  ic=0  mode=Unused parameter value
      settings: LibrarySourceBlock=commsequence2/Repeat
  T_cleanup4 : Terminator
  T_cleanup5 : Terminator
  Terminator{,1..3} (4 alike) : Terminator
  dataOutI : Outport
  dataOutQ : Outport  Port=2
  validOut : Outport  Port=3
  extWordPop : Outport  Port=4
  fs_txur : Outport  Port=5
  wires:
  Delay5/1 -> dataOutI/1
  Delay7/1 -> Delay5/1
  Delay3/1 -> validOut/1
  Cast To Boolean/1 -> Delay7/1
  Complex to Real-Imag/2 -> Cast To Boolean1/1
  Complex to Real-Imag/1 -> Cast To Boolean/1
  Delay8/1 -> Delay4/1
  Repeat/1 -> Delay9/1
  Delay4/1 -> dataOutQ/1
  Repeat2/1 -> Complex to Real-Imag/1
  Delay2/1 -> AND/2
  Bit Slice1/1 -> Data Type Conversion1/1
  Input Data/2(txValid) -> QPSK Tx/2(validIn)
  Downsample/1 -> Terminator3/1
  Bit Slice/1 -> Delay2/1
  Delay1/1 -> Bit Slice1/1, Bit Slice/1
  Input Data/5(fs_txur) -> fs_txur/1
  extWord/1 -> Input Data/3(extWord)
  dataQ/1 -> Downsample2/1
  Downsample3/1 -> Terminator2/1
  Constant/1 -> Delay1/1
  Cast To Boolean1/1 -> Delay8/1
  Downsample2/1 -> Terminator1/1
  debug/1 -> Downsample/1
  QPSK Tx/1(dataReady) -> Delay/1
  validIn/1 -> Downsample3/1
  Downsample1/1 -> Terminator/1
  dataI/1 -> Downsample1/1
  Input Data/4(extWordPop) -> extWordPop/1
  QPSK Tx/4(validOut) -> Repeat/1
  Data Type Conversion1/1 -> Input Data/2(reset)
  Delay9/1 -> Delay3/1
  Input Data/3(msg_count_out) -> Repeat1/1
  extWordAvail/1 -> Input Data/4(extWordAvail)
  AND/1 -> Input Data/1(enb)
  extWordFirst/1 -> Input Data/6(extWordFirst)
  Data Type Conversion/1 -> QPSK Tx/1(dataIn)
  Delay/1 -> AND/1
  Input Data/1(txData) -> Data Type Conversion/1
  extBitSel/1 -> Input Data/5(extBitSel)
  QPSK Tx/2(dataOut) -> Repeat2/1
  QPSK Tx/3(txDiagBus) -> T_cleanup4/1
  Repeat1/1 -> T_cleanup5/1

== system commhdlQPSKTxRxLoopback/Receiver/QPSK Rx/Automatic Gain Control ==
  dataIn : Inport
  validIn : Inport  Port=2
  Data Type Conversion : DataTypeConversion  OutDataTypeStr=fixdt(1,16,10)  SaturateOnIntegerOverflow=off  RndMeth=Floor
  Delay{1..5} (5 alike) : Delay
  Error Detector : Subsystem
  Loop Filter : Subsystem
  Product : Product  OutDataTypeStr=Inherit: Same as first input
  dataOut : Outport
  validOut : Outport  Port=2
  wires:
  Data Type Conversion/1 -> Delay1/1
  Delay5/1 -> Delay3/1
  Delay3/1 -> validOut/1
  Delay4/1 -> Product/1
  Delay1/1 -> Product/2
  Loop Filter/1(gain) -> Data Type Conversion/1
  Error Detector/1(err) -> Loop Filter/1(err)
  validIn/1 -> Delay5/1
  Delay2/1 -> Error Detector/1(dataIn), dataOut/1
  dataIn/1 -> Delay4/1
  Product/1 -> Delay2/1

== system commhdlQPSKTxRxLoopback/Receiver/QPSK Rx/Frequency and Time Synchronizer ==
  dataIn : Inport
  validIn : Inport  Port=2
  rstCS : Inport  Port=3
  Carrier Synchronizer : Subsystem
      settings: PortSchema="{\"entries\":[{\"content\":{\"sides\":[{\"content\":{\"connectorIds\":[\"In1\",\"In2\",\"In3\"]},\"type\":\"ConnectorPlacement.EquallySpacedRectSide\",\"uuid\":\"ee58e5dc-083a-48cb-b7f3-66ed8a15890f\"},{\"content\":{\"connectorIds\":[\"Out1\",\"Out2\"],\"side\":\"RIGHT\"},\"type\":\"ConnectorPlacement.EquallySpacedRectSide\",\"uuid\":\"6d121164-5065-4840-a82e-fa57a8e9650e\"},{\"content\":{\"connectorIds\":[\"In4\"],\"side\":\"TOP\"},\"type\":\"ConnectorPlacement.EquallySpacedRectSide\",\"uuid\":\"54d2b8e3-f516-4572-94a0-c914196ae8e4\"}]},\"type\":\"ConnectorPlacement.EquallySpacedConnector\",\"uuid\":\"0f2a6472-efd0-42ca-a030-ab436081b5e1\"}],\"packageUris\":[\"http://schema.mathworks.com/mf0/Connector/R2020b\"],\"version\":\"1.0\"}"
  Coarse Frequency Compensator : Subsystem
      settings: PortSchema="{\"entries\":[{\"content\":{\"sides\":[{\"content\":{\"connectorIds\":[\"In1\",\"In2\"]},\"type\":\"ConnectorPlacement.EquallySpacedRectSide\",\"uuid\":\"138aa5bd-62db-47d6-b55f-f529a6004434\"},{\"content\":{\"connectorIds\":[\"Out1\",\"Out2\",\"Out3\"],\"side\":\"RIGHT\"},\"type\":\"ConnectorPlacement.EquallySpacedRectSide\",\"uuid\":\"8e6ccec0-f736-48ab-be6d-feac886e083d\"},{\"content\":{\"connectorIds\":[\"Out4\"],\"side\":\"TOP\"},\"type\":\"ConnectorPlacement.EquallySpacedRectSide\",\"uuid\":\"d4535392-74fa-432a-a39c-b98ba26e8163\"},{\"content\":{\"side\":\"BOTTOM\"},\"type\":\"ConnectorPlacement.EquallySpacedRectSide\",\"uuid\":\"770ac6a2-7a02-4a77-858b-592982deaf6e\"}]},\"type\":\"ConnectorPlacement.EquallySpacedConnector\",\"uuid\":\"a9b944be-f88b-4ab6-a5e1-6824362eb9ca\"}],\"packageUris\":[\"http://schema.mathworks.com/mf0/Connector/R2020b\"],\"version\":\"1.0\"}"
  No HDL : Subsystem
      settings: PortSchema="{\"entries\":[{\"content\":{\"sides\":[{\"content\":{\"connectorIds\":[\"In1\",\"In2\"]},\"type\":\"ConnectorPlacement.EquallySpacedRectSide\",\"uuid\":\"df96a46d-149f-4580-adf6-e5cf26cffa9b\"},{\"content\":{\"connectorIds\":[\"In3\",\"In4\"],\"side\":\"RIGHT\"},\"type\":\"ConnectorPlacement.EquallySpacedRectSide\",\"uuid\":\"1c46d09c-cb37-4618-ac4e-e5ef50df41fb\"},{\"content\":{\"connectorIds\":[],\"side\":\"TOP\"},\"type\":\"ConnectorPlacement.EquallySpacedRectSide\",\"uuid\":\"7fe62300-46d7-4234-a31d-eecffed4f6e6\"},{\"content\":{\"connectorIds\":[],\"side\":\"BOTTOM\"},\"type\":\"ConnectorPlacement.EquallySpacedRectSide\",\"uuid\":\"05ecd563-28f5-4cfd-b718-5032a7458763\"}]},\"type\":\"ConnectorPlacement.EquallySpacedConnector\",\"uuid\":\"4b3d5859-a469-4389-9e5d-e5f07416a9a1\"}],\"packageUris\":[\"http://schema.mathworks.com/mf0/Connector/R2020b\"],\"version\":\"1.0\"}"
  Packet Controller : Subsystem
  Phase Ambiguity Estimation and Correction : Subsystem
  Preamble Detector : Subsystem
  Symbol Synchronizer : Subsystem
  dataOut : Outport
  startOut : Outport  Port=2
  endOut : Outport  Port=3
  validOut : Outport  Port=4
  postSymbolSync : Outport  Port=5
  postCarrierSync : Outport  Port=6
  nSynced : Outport  Port=7
  normCoarseFreqEst : Outport  Port=8
  wires:
  Coarse Frequency Compensator/3(validOut) -> Carrier Synchronizer/3(validIn)
  Coarse Frequency Compensator/1(dataOut) -> Carrier Synchronizer/1(dataIn)
  Phase Ambiguity Estimation and Correction/1(dataOut) -> Packet Controller/1(dataIn)
  Phase Ambiguity Estimation and Correction/3(validOut) -> Packet Controller/3(validIn)
  Symbol Synchronizer/2(validOut) -> No HDL/2(In2), Coarse Frequency Compensator/2(validIn)
  Symbol Synchronizer/1(dataOut) -> postSymbolSync/1, No HDL/1(In1), Coarse Frequency Compensator/1(dataIn)
  Phase Ambiguity Estimation and Correction/2(syncPulseOut) -> Packet Controller/2(syncPulse)
  Preamble Detector/3(validOut) -> Phase Ambiguity Estimation and Correction/3(validIn)
  Preamble Detector/1(dataOut) -> Phase Ambiguity Estimation and Correction/1(dataIn)
  validIn/1 -> Symbol Synchronizer/2(validIn)
  dataIn/1 -> Symbol Synchronizer/1(dataIn)
  Coarse Frequency Compensator/2(rstCS) -> Carrier Synchronizer/2(internalRst)
  Packet Controller/1(dataOut) -> dataOut/1
  Packet Controller/2(startOut) -> startOut/1
  Packet Controller/3(endOut) -> endOut/1
  Packet Controller/4(validOut) -> validOut/1
  Preamble Detector/2(syncPulse) -> nSynced/1, Phase Ambiguity Estimation and Correction/2(syncPulseIn)
  Carrier Synchronizer/1(dataOut) -> postCarrierSync/1, No HDL/3(In3), Preamble Detector/1(dataIn)
  Carrier Synchronizer/2(validOut) -> No HDL/4(In4), Preamble Detector/2(validIn)
  Coarse Frequency Compensator/4(normalizedFreqEst) -> normCoarseFreqEst/1
  rstCS/1 -> Carrier Synchronizer/4(manualRst)

== system commhdlQPSKTxRxLoopback/Receiver/QPSK Rx/HDL Data Descrambler ==
  note: HDL Data Scrambler
      | Polynomial: x^7+x^4+1
      | Initial state: [1 0 1 1 1 0 1]
  dataIn : Inport
  startIn : Inport  Port=2
  endIn : Inport  Port=3
  validIn : Inport  Port=4
  BIT_XOR : Logic  Operator=XOR  IconShape=distinctive  AllPortsSameDT=off  OutDataTypeStr=boolean
  BIT_XOR2 : Logic  Operator=XOR  IconShape=distinctive  AllPortsSameDT=off  OutDataTypeStr=boolean
  Delay{,1..7} (8 alike) : Delay  DelayLength=1
  EnableScrambling : Constant  Value=true  SampleTime=-1
  Logical Operator : Logic  IconShape=distinctive  AllPortsSameDT=off  OutDataTypeStr=boolean
  Switch : Switch  Criteria=u2 > Threshold  SaturateOnIntegerOverflow=off  InputSameDT=off
  Unit Delay Enabled Resettable Synchronous{,2..3,5,7} (5 alike) : hdlsllib/Discrete/Unit Delay Enabled Resettable Synchronous  InitialCondition=1  SampleTime=-1
  Unit Delay Enabled Resettable Synchronous1 : hdlsllib/Discrete/Unit Delay Enabled Resettable Synchronous  InitialCondition=0  SampleTime=-1
  Unit Delay Enabled Resettable Synchronous4 : hdlsllib/Discrete/Unit Delay Enabled Resettable Synchronous  InitialCondition=0  SampleTime=-1
  Unit Delay Enabled Resettable Synchronous6 : hdlsllib/Discrete/Unit Delay Enabled Resettable Synchronous  InitialCondition=0.0  SampleTime=-1
  dataOut : Outport  InitialOutput=0
  startOut : Outport  Port=2  InitialOutput=0
  endOut : Outport  Port=3  InitialOutput=0
  validOut : Outport  Port=4  InitialOutput=0
  wires:
  Delay4/1 -> validOut/1
  Delay3/1 -> dataOut/1
  endIn/1 -> Delay2/1, Unit Delay Enabled Resettable Synchronous4/3
  Logical Operator/1 -> BIT_XOR2/2
  Unit Delay Enabled Resettable Synchronous4/1 -> Logical Operator/1
  Delay1/1 -> Unit Delay Enabled Resettable Synchronous6/2, Unit Delay Enabled Resettable Synchronous2/2, Unit Delay Enabled Resettable Synchronous1/2, Unit Delay Enabled Resettable Synchronous/2, Delay4/1, Unit Delay Enabled Resettable Synchronous3/2, Unit Delay Enabled Resettable Synchronous5/2, Unit Delay Enabled Resettable Synchronous7/2
  Delay/1 -> Switch/3, BIT_XOR2/1
  startIn/1 -> Delay5/1, Unit Delay Enabled Resettable Synchronous4/1, Unit Delay Enabled Resettable Synchronous4/2, Unit Delay Enabled Resettable Synchronous6/3, Unit Delay Enabled Resettable Synchronous5/3, Unit Delay Enabled Resettable Synchronous1/3, Unit Delay Enabled Resettable Synchronous/3, Unit Delay Enabled Resettable Synchronous2/3, Unit Delay Enabled Resettable Synchronous3/3, Unit Delay Enabled Resettable Synchronous7/3
  dataIn/1 -> Delay/1
  validIn/1 -> Delay1/1
  BIT_XOR/1 -> Unit Delay Enabled Resettable Synchronous/1, Logical Operator/2
  Unit Delay Enabled Resettable Synchronous1/1 -> Unit Delay Enabled Resettable Synchronous2/1
  Unit Delay Enabled Resettable Synchronous2/1 -> Unit Delay Enabled Resettable Synchronous3/1
  Unit Delay Enabled Resettable Synchronous/1 -> Unit Delay Enabled Resettable Synchronous1/1
  Unit Delay Enabled Resettable Synchronous3/1 -> BIT_XOR/2, Unit Delay Enabled Resettable Synchronous5/1
  Unit Delay Enabled Resettable Synchronous5/1 -> Unit Delay Enabled Resettable Synchronous6/1
  Unit Delay Enabled Resettable Synchronous6/1 -> Unit Delay Enabled Resettable Synchronous7/1
  Unit Delay Enabled Resettable Synchronous7/1 -> BIT_XOR/1
  Delay2/1 -> Delay6/1
  Delay5/1 -> Delay7/1
  Delay6/1 -> endOut/1
  Delay7/1 -> startOut/1
  EnableScrambling/1 -> Switch/2
  BIT_XOR2/1 -> Switch/1
  Switch/1 -> Delay3/1

== system commhdlQPSKTxRxLoopback/Receiver/QPSK Rx/QPSK Demodulator ==
  dataIn : Inport
  startIn : Inport  Port=2
  endIn : Inport  Port=3
  validIn : Inport  Port=4
  Delay{,1..13} (14 alike) : Delay  DelayLength=1
  QPSK Demodulator Baseband : commdigbbndpm3/QPSK Demodulator Baseband  OutType=Bit  DecType=Hard decision  VarSource=Dialog  Variance=1  Dec=Gray  Ph=pi/4  outDtype1=boolean  outDtype2=Inherit via internal rule  derotateFactorWordLen=16  derotateFactorDataTypeStr=Inherit: Same word length as input  derotateFactorLastDataTypeStr=Inherit: Same word length as input
  Serializer : Subsystem
  Signal Specification : SignalSpecification  Dimensions=1
  dataOut : Outport
  startOut : Outport  Port=2
  endOut : Outport  Port=3
  validOut : Outport  Port=4
  wires:
  Delay/1 -> QPSK Demodulator Baseband/1
  Delay1/1 -> Delay5/1
  Delay6/1 -> Delay4/1
  Delay7/1 -> Delay13/1
  Delay2/1 -> Delay6/1
  Delay3/1 -> Delay7/1
  Signal Specification/1 -> Delay/1
  QPSK Demodulator Baseband/1 -> Delay12/1
  Delay8/1 -> dataOut/1
  Delay9/1 -> validOut/1
  Delay10/1 -> startOut/1
  Delay11/1 -> endOut/1
  Delay5/1 -> Serializer/2(In2)
  Delay12/1 -> Serializer/1(u)
  Delay4/1 -> Delay10/1
  Delay13/1 -> Delay11/1
  Serializer/1(Out1) -> Delay8/1
  Serializer/2(Out2) -> Delay9/1
  dataIn/1 -> Signal Specification/1
  validIn/1 -> Delay1/1
  startIn/1 -> Delay2/1
  endIn/1 -> Delay3/1
